simulink model "bldc_6step_speed"  (R2024b)
settings: Solver=ode45  StartTime=0.0  StopTime=0.5  FixedStep=1e-6  MaxStep=1e-6  RelTol=1e-3
libraries: simulink x1, slpidlib x1
settings Model: Creator=mehme  LastModifiedBy=mehme

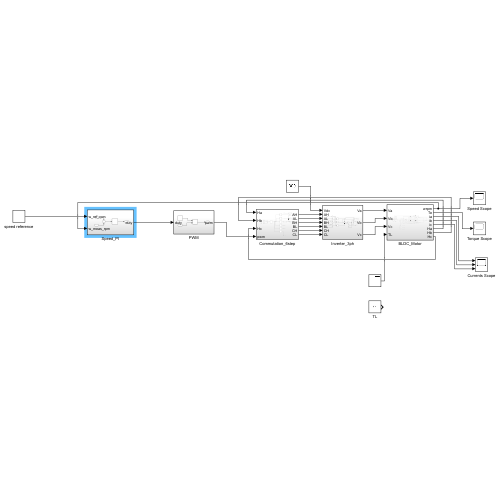
[thumbnail: Simulink's stored preview of the top-level diagram]
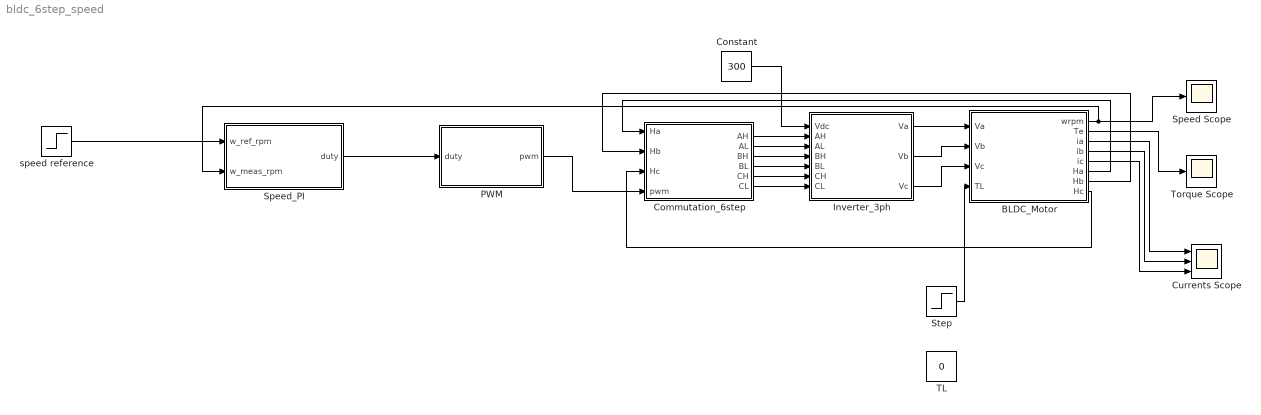
== system bldc_6step_speed ==
  BLDC_Motor : Subsystem
  Commutation_6step : Subsystem
  Constant : Constant  Value=300
  Currents Scope : Scope  NumInputPorts=3
  Inverter_3ph : Subsystem
  PWM : Subsystem
  Speed Scope : Scope
  Speed_PI : Subsystem
  Step : Step  Time=0.2  After=3  SampleTime=0
  TL : Constant  Value=0
  Torque Scope : Scope
  speed reference : Step  Time=0  Before=2000  After=2000  SampleTime=0
  wires:
  Speed_PI/1(duty) -> PWM/1(duty)
  Commutation_6step/1(AH) -> Inverter_3ph/2(AH)
  Commutation_6step/2(AL) -> Inverter_3ph/3(AL)
  Commutation_6step/3(BH) -> Inverter_3ph/4(BH)
  Commutation_6step/4(BL) -> Inverter_3ph/5(BL)
  Commutation_6step/5(CH) -> Inverter_3ph/6(CH)
  Commutation_6step/6(CL) -> Inverter_3ph/7(CL)
  Constant/1 -> Inverter_3ph/1(Vdc)
  BLDC_Motor/6(Ha) -> Commutation_6step/1(Ha)
  BLDC_Motor/7(Hb) -> Commutation_6step/2(Hb)
  BLDC_Motor/8(Hc) -> Commutation_6step/3(Hc)
  PWM/1(pwm) -> Commutation_6step/4(pwm)
  Inverter_3ph/1(Va) -> BLDC_Motor/1(Va)
  Inverter_3ph/2(Vb) -> BLDC_Motor/2(Vb)
  Inverter_3ph/3(Vc) -> BLDC_Motor/3(Vc)
  speed reference/1 -> Speed_PI/1(w_ref_rpm)
  BLDC_Motor/1(wrpm) -> Speed Scope/1, Speed_PI/2(w_meas_rpm)
  BLDC_Motor/2(Te) -> Torque Scope/1
  BLDC_Motor/3(ia) -> Currents Scope/1
  BLDC_Motor/4(ib) -> Currents Scope/2
  BLDC_Motor/5(ic) -> Currents Scope/3
  Step/1 -> BLDC_Motor/4(TL)

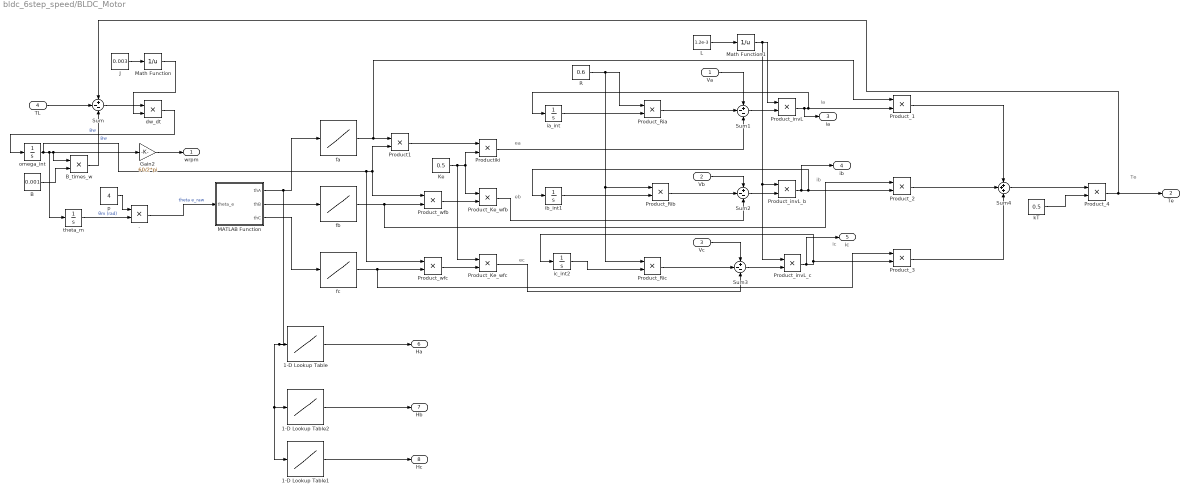
== system bldc_6step_speed/BLDC_Motor ==
  note: Te
  note: ic
  note: ib
  note: ia
  note: ec
  note: ea
  note: eb
  Va : Inport
  Vb : Inport  Port=2
  Vc : Inport  Port=3
  TL : Inport  Port=4
  . : Product
  1-D Lookup Table : Lookup_n-D  NumberOfTableDimensions=1  BreakpointsForDimension1=[0 pi/3 2*pi/3 pi 4*pi/3 5*pi/3 2*pi]  Table=[0 1 1 1 0 0 0]  InternalRulePriority=Speed  RndMeth=Simplest
  1-D Lookup Table1 : Lookup_n-D  NumberOfTableDimensions=1  BreakpointsForDimension1=[0 pi/3 2*pi/3 pi 4*pi/3 5*pi/3 2*pi]  Table=[1 1 0 0 0 1 1]  InternalRulePriority=Speed  RndMeth=Simplest
  1-D Lookup Table2 : Lookup_n-D  NumberOfTableDimensions=1  BreakpointsForDimension1=[0 pi/3 2*pi/3 pi 4*pi/3 5*pi/3 2*pi]  Table=[0 0 0 1 1 1 1]  InternalRulePriority=Speed  RndMeth=Simplest
  B : Constant  Value=0.001
  B_times_w : Product
  Gain2 : Gain  Gain=60/2*pi
  J : Constant  Value=0.003
  Ke : Constant  Value=0.5
  L : Constant  Value=1.2e-3
  MATLAB Function : MATLAB Function  TreatAsAtomicUnit=on
  Math Function : Math  Operator=reciprocal
  Math Function1 : Math  Operator=reciprocal
  Product1 : Product
  Product_{1..4} (4 alike) : Product
  Product_Ke_wfb : Product
  Product_Ke_wfc : Product
  Product_Ria : Product
  Product_Rib : Product
  Product_Ric : Product
  Product_invL : Product
  Product_invL_b : Product
  Product_invL_c : Product
  Product_wfb : Product
  Product_wfc : Product
  Productiki : Product
  R : Constant  Value=0.6
  Sum{,1..3} (4 alike) : Sum  Inputs=+--
  Sum4 : Sum  Inputs=+++
  dw_dt : Product
  fa : Lookup_n-D  NumberOfTableDimensions=1  BreakpointsForDimension1=[0 pi/3 pi 4*pi/3 2*pi]  Table=[-1 1 1 -1 -1]  InternalRulePriority=Speed  RndMeth=Simplest
  fb : Lookup_n-D  NumberOfTableDimensions=1  BreakpointsForDimension1=[0 pi/3 pi 4*pi/3 2*pi]  Table=[-1 1 1 -1 -1]  InternalRulePriority=Speed  RndMeth=Simplest
  fc : Lookup_n-D  NumberOfTableDimensions=1  BreakpointsForDimension1=[0 pi/3 pi 4*pi/3 2*pi]  Table=[-1 1 1 -1 -1]  InternalRulePriority=Speed  RndMeth=Simplest
  ia_int : Integrator
  ib_int1 : Integrator
  ic_int2 : Integrator
  kT : Constant  Value=0.5
  omega_int : Integrator
  p : Constant  Value=4
  theta_m : Integrator
  wrpm : Outport
  Te : Outport  Port=2
  ia : Outport  Port=3
  ib : Outport  Port=4
  ic : Outport  Port=5
  Ha : Outport  Port=6
  Hb : Outport  Port=7
  Hc : Outport  Port=8
  wires:
  TL/1 -> Sum/2
  Sum/1 -> dw_dt/1
  Gain2/1 -> wrpm/1
  B/1 -> B_times_w/2
  B_times_w/1 -> Sum/3  "Bw"
  J/1 -> Math Function/1
  Math Function/1 -> dw_dt/2
  dw_dt/1 -> omega_int/1  "Bw"
  p/1 -> ./1
  theta_m/1 -> ./2  "θm (rad)"
  ./1 -> MATLAB Function/1(theta_e)  "theta e_raw"
  MATLAB Function/1(thA) -> 1-D Lookup Table1/1, 1-D Lookup Table2/1, 1-D Lookup Table/1, fa/1
  MATLAB Function/2(thB) -> fb/1
  MATLAB Function/3(thC) -> fc/1
  L/1 -> Math Function1/1
  fa/1 -> Product_1/1, Product1/1
  omega_int/1 -> Product_wfc/1, Product1/2, Product_wfb/1, theta_m/1, Gain2/1, B_times_w/1
  Product1/1 -> Productiki/1
  Ke/1 -> Product_Ke_wfc/1, Productiki/2, Product_Ke_wfb/1
  Va/1 -> Sum1/1
  fb/1 -> Product_2/1, Product_wfb/2
  Product_wfb/1 -> Product_Ke_wfb/2
  fc/1 -> Product_3/1, Product_wfc/2
  Product_wfc/1 -> Product_Ke_wfc/2
  R/1 -> Product_Ric/1, Product_Rib/1, Product_Ria/1
  ia_int/1 -> Product_Ria/2
  Product_Ria/1 -> Sum1/2
  Productiki/1 -> Sum1/3
  Sum1/1 -> Product_invL/2
  Math Function1/1 -> Product_invL_c/1, Product_invL_b/1, Product_invL/1
  Product_invL/1 -> ia/1, Product_1/2, ia_int/1
  ib_int1/1 -> Product_Rib/2
  Vb/1 -> Sum2/1
  Product_Rib/1 -> Sum2/2
  Product_Ke_wfb/1 -> Sum2/3
  Sum2/1 -> Product_invL_b/2
  Product_invL_b/1 -> ib/1, ib_int1/1, Product_2/2
  Vc/1 -> Sum3/1
  Product_Ric/1 -> Sum3/2
  ic_int2/1 -> Product_Ric/2
  Product_Ke_wfc/1 -> Sum3/3
  Sum3/1 -> Product_invL_c/2
  Product_invL_c/1 -> ic/1, ic_int2/1, Product_3/2
  Product_1/1 -> Sum4/1
  Product_2/1 -> Sum4/2
  Product_3/1 -> Sum4/3
  Sum4/1 -> Product_4/1
  kT/1 -> Product_4/2
  Product_4/1 -> Te/1, Sum/1
  1-D Lookup Table/1 -> Ha/1
  1-D Lookup Table2/1 -> Hb/1
  1-D Lookup Table1/1 -> Hc/1

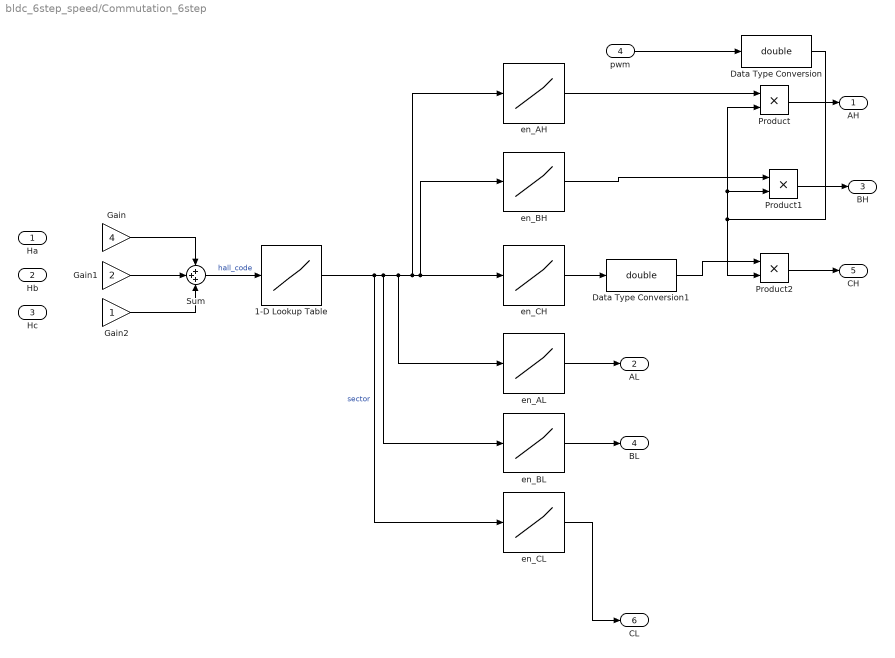
== system bldc_6step_speed/Commutation_6step ==
  Ha : Inport
  Hb : Inport  Port=2
  Hc : Inport  Port=3
  pwm : Inport  Port=4
  1-D Lookup Table : Lookup_n-D  NumberOfTableDimensions=1  BreakpointsForDimension1=[1 2 3 4 5 6]  Table=[1 5 6 3 2 4]  InternalRulePriority=Speed  RndMeth=Simplest
  Data Type Conversion : DataTypeConversion  OutDataTypeStr=double  SaturateOnIntegerOverflow=off  RndMeth=Floor
  Data Type Conversion1 : DataTypeConversion  OutDataTypeStr=double  SaturateOnIntegerOverflow=off  RndMeth=Floor
  Gain : Gain  Gain=4
  Gain1 : Gain  Gain=2
  Gain2 : Gain
  Product : Product
  Product1 : Product
  Product2 : Product
  Sum : Sum  Inputs=+++
  en_AH : Lookup_n-D  NumberOfTableDimensions=1  BreakpointsForDimension1=[1 2 3 4 5 6]  Table=[1 1 0 0 0 0]  InternalRulePriority=Speed  RndMeth=Simplest
  en_AL : Lookup_n-D  NumberOfTableDimensions=1  BreakpointsForDimension1=[1 2 3 4 5 6]  Table=[0 0 0 1 1 0]  InternalRulePriority=Speed  RndMeth=Simplest
  en_BH : Lookup_n-D  NumberOfTableDimensions=1  BreakpointsForDimension1=[1 2 3 4 5 6]  Table=[0 0 1 1 0 0]  InternalRulePriority=Speed  RndMeth=Simplest
  en_BL : Lookup_n-D  NumberOfTableDimensions=1  BreakpointsForDimension1=[1 2 3 4 5 6]  Table=[1 0 0 0 0 1]  InternalRulePriority=Speed  RndMeth=Simplest
  en_CH : Lookup_n-D  NumberOfTableDimensions=1  BreakpointsForDimension1=[1 2 3 4 5 6]  Table=[0 0 0 0 1 1]  InternalRulePriority=Speed  RndMeth=Simplest
  en_CL : Lookup_n-D  NumberOfTableDimensions=1  BreakpointsForDimension1=[1 2 3 4 5 6]  Table=[0 1 1 0 0 0]  InternalRulePriority=Speed  RndMeth=Simplest
  AH : Outport
  AL : Outport  Port=2
  BH : Outport  Port=3
  BL : Outport  Port=4
  CH : Outport  Port=5
  CL : Outport  Port=6
  wires:
  Gain/1 -> Sum/1
  Gain1/1 -> Sum/2
  Gain2/1 -> Sum/3
  Sum/1 -> 1-D Lookup Table/1  "hall_code"
  1-D Lookup Table/1 -> en_CL/1, en_BL/1, en_AL/1, en_AH/1, en_BH/1, en_CH/1  "sector"
  Product/1 -> AH/1
  en_AH/1 -> Product/1
  Data Type Conversion/1 -> Product/2, Product1/2, Product2/2
  en_BH/1 -> Product1/1
  Product1/1 -> BH/1
  Product2/1 -> CH/1
  en_AL/1 -> AL/1
  en_BL/1 -> BL/1
  en_CL/1 -> CL/1
  pwm/1 -> Data Type Conversion/1
  en_CH/1 -> Data Type Conversion1/1
  Data Type Conversion1/1 -> Product2/1

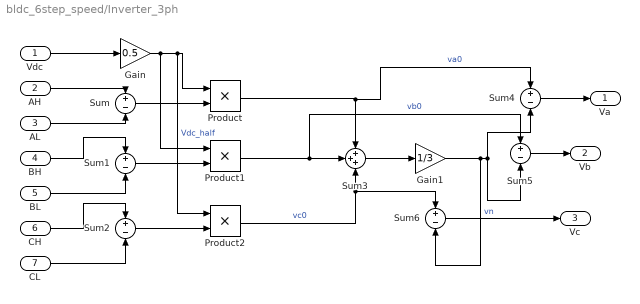
== system bldc_6step_speed/Inverter_3ph ==
  Vdc : Inport
  AH : Inport  Port=2
  AL : Inport  Port=3
  BH : Inport  Port=4
  BL : Inport  Port=5
  CH : Inport  Port=6
  CL : Inport  Port=7
  Gain : Gain  Gain=0.5
  Gain1 : Gain  Gain=1/3
  Product : Product
  Product1 : Product
  Product2 : Product
  Sum{,1..2,4..6} (6 alike) : Sum  Inputs=+-
  Sum3 : Sum  Inputs=+++
  Va : Outport
  Vb : Outport  Port=2
  Vc : Outport  Port=3
  wires:
  Vdc/1 -> Gain/1
  AH/1 -> Sum/1
  AL/1 -> Sum/2
  BL/1 -> Sum1/2
  BH/1 -> Sum1/1
  CH/1 -> Sum2/1
  CL/1 -> Sum2/2
  Sum/1 -> Product/2
  Gain/1 -> Product1/1, Product2/1, Product/1  "Vdc_half"
  Sum1/1 -> Product1/2
  Sum2/1 -> Product2/2
  Product1/1 -> Sum5/1, Sum3/2  "vb0"
  Product/1 -> Sum4/1, Sum3/1  "va0"
  Product2/1 -> Sum6/1, Sum3/3  "vc0"
  Sum3/1 -> Gain1/1
  Gain1/1 -> Sum6/2, Sum4/2, Sum5/2  "vn"
  Sum6/1 -> Vc/1
  Sum5/1 -> Vb/1
  Sum4/1 -> Va/1

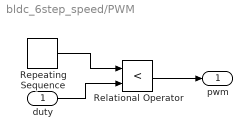
== system bldc_6step_speed/PWM ==
  duty : Inport
  Relational Operator : RelationalOperator  Operator=<  OutDataTypeStr=boolean  RndMeth=Simplest  InputSameDT=off
  Repeating Sequence : simulink/Sources/Repeating Sequence  rep_seq_t=[0 5e-5 1e-4]  rep_seq_y=[0 1 0]
  pwm : Outport
  wires:
  Repeating Sequence/1 -> Relational Operator/1
  duty/1 -> Relational Operator/2
  Relational Operator/1 -> pwm/1

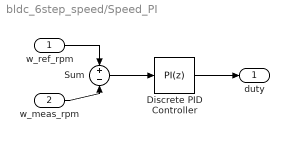
== system bldc_6step_speed/Speed_PI ==
  w_ref_rpm : Inport
  w_meas_rpm : Inport  Port=2
  Discrete PID Controller : slpidlib/PID Controller  Controller=PI  Form=Parallel  TimeDomain=Discrete-time  UseExternalTs=off  SampleTime=1e-4  IntegratorMethod=Forward Euler  FilterMethod=Forward Euler  ControllerParametersSource=internal  P=0.0005  I=0.05  UseKiTs=off  D=0  UseExternalDerivativeSource=off  N=100  UseFilter=on  TunerSelectOption=Transfer Function Based (PID Tuner App)  InitialConditionSource=internal  InitialConditionForIntegrator=0  InitialConditionForFilter=0  DifferentiatorICPrevScaledInput=0  ExternalReset=none  TrackingMode=off  Kt=1  LimitOutput=on  SatLimitsSource=internal  UpperSaturationLimit=0.95  LowerSaturationLimit=0  LinearizeAsGain=off  AntiWindupMode=back-calculation  Kb=1  LimitIntegrator=off  UpperIntegratorSaturationLimit=inf  LowerIntegratorSaturationLimit=-inf  POutMin=[]  POutMax=[]  IOutMin=[]  IOutMax=[]  DOutMin=[]  DOutMax=[]  NOutMin=[]  NOutMax=[]  SumOutMin=[]  SumOutMax=[]  SaturationOutMin=[]  SaturationOutMax=[]  PParamMin=[]  PParamMax=[]  IParamMin=[]  IParamMax=[]  DParamMin=[]  DParamMax=[]  NParamMin=[]  NParamMax=[]  KbParamMin=[]  KbParamMax=[]  KtParamMin=[]  KtParamMax=[]  KbOutMin=[]  KbOutMax=[]  KtOutMin=[]  KtOutMax=[]  IntegratorOutMin=[]  IntegratorOutMax=[]  FilterOutMin=[]  FilterOutMax=[]  SumI1OutMin=[]  SumI1OutMax=[]  SumI2OutMin=[]  SumI2OutMax=[]  SumI3OutMin=[]  SumI3OutMax=[]  SumI4OutMin=[]  SumI4OutMax=[]  SumDOutMin=[]  SumDOutMax=[]  DifferentiatorOutMin=[]  DifferentiatorOutMax=[]  FilterDiffOutCoefMin=[]  FilterDiffOutCoefMax=[]  ReciprocalOutMin=[]  ReciprocalOutMax=[]  SumDenOutMin=[]  SumDenOutMax=[]  SumNumOutMin=[]  SumNumOutMax=[]  DivideOutMin=[]  DivideOutMax=[]  UdiffTsProdOutMin=[]  UdiffTsProdOutMax=[]  NTsProdOutMin=[]  NTsProdOutMax=[]  UintegralTsProdOutMin=[]  UintegralTsProdOutMax=[]  UngainTsProdOutMin=[]  UngainTsProdOutMax=[]  ClampingZeroOutDataTypeStr=Inherit: Inherit via back propagation  ClampingZeroOutMin=[]  ClampingZeroOutMax=[]  FilterDenConstantOutDataTypeStr=Inherit: Inherit via back propagation  FilterDenConstantOutMin=[]  FilterDenConstantOutMax=[]  PCopyOutDataTypeStr=Inherit: Inherit via back propagation  PCopyOutMin=[]  PCopyOutMax=[]  NCopyOutDataTypeStr=Inherit: Inherit via back propagation  NCopyOutMin=[]  NCopyOutMax=[]  IntegratorContinuousStateAttributes=''  IntegratorStateMustResolveToSignalObject=off  IntegratorRTWStateStorageClass=Auto  FilterContinuousStateAttributes=''  FilterStateMustResolveToSignalObject=off  FilterRTWStateStorageClass=Auto  ParallelPVariant=InternalParameters  IdealPVariant=Disabled  IVariant=InternalParameters  DVariant=Disabled  IntegratorVariant=Discrete  SatVariant=Enabled  AWVariant=BackCalculation  PCopyVariant=Disabled  TRVariant=Disabled  FdbkBlocksVariant=Forward  IdealPFdbkVariant=Disabled  SatFdbkVariant=Disabled  DerivativeFilterVariant=Disabled  NVariant=Disabled  NCopyVariant=Disabled_SignalSpec  FilterICVariant=Disabled  IntegratorICVariant=InternalICs  ExternalResetVariant=Disabled  TRSumVariant=Passthrough  SumFdbkVariant=Disabled  SumVariant=Sum_PI  TsampFilterVariant=InternalTs  TsampNgainVariant=Passthrough  TsampIntegralVariant=Disabled_SignalSpec  ExternalSaturationOutDataTypeStr=Inherit: Same as second input  DerivativeSourceVariant=Disabled  PreIntVariant=InternalPreInt
      settings: LibrarySourceBlock=simulink/Discrete/Discrete PID Controller
  Sum : Sum  Inputs=+-
  duty : Outport
  wires:
  w_ref_rpm/1 -> Sum/1
  w_meas_rpm/1 -> Sum/2
  Sum/1 -> Discrete PID Controller/1
  Discrete PID Controller/1 -> duty/1

== matlab function bldc_6step_speed/BLDC_Motor/MATLAB Function ==
  data: theta_e input; thA output; thB output; thC output
function [thA, thB, thC] = wrap_angles(theta_e)
twoPi = 2*pi;
thA = mod(theta_e, twoPi);
thB = mod(theta_e - 2*pi/3, twoPi);
thC = mod(theta_e + 2*pi/3, twoPi);
end
